simulink model "nms_sim_2D_cost"  (R2024b)
settings: Solver=ode15s  StartTime=0.0  StopTime=t_sim  MaxStep=dt_max  EnableMultiTasking=on
values from neighbouring files (symbols this model uses):
  a_BFSH = param_ctrl(35)*1    [setCtrlPar_optim_CPGreflex2001_2D.m]
  a_GAS = param_ctrl(37)*1    [setCtrlPar_optim_CPGreflex2001_2D.m]
  a_GLU = param_ctrl(31)*1    [setCtrlPar_optim_CPGreflex2001_2D.m]
  a_HAM = param_ctrl(33)*1    [setCtrlPar_optim_CPGreflex2001_2D.m]
  a_HFL = param_ctrl(32)*1    [setCtrlPar_optim_CPGreflex2001_2D.m]
  a_RF = param_ctrl(34)*1    [setCtrlPar_optim_CPGreflex2001_2D.m]
  a_SOL = param_ctrl(38)*1    [setCtrlPar_optim_CPGreflex2001_2D.m]
  a_TA = param_ctrl(39)*1    [setCtrlPar_optim_CPGreflex2001_2D.m]
  a_VAS = param_ctrl(36)*1    [setCtrlPar_optim_CPGreflex2001_2D.m]
  ai = param_ctrl(96)*2.0    [setCtrlPar_optim_CPGreflex2001_2D.m]
  b_BFSH = param_ctrl(52)*.51    [setCtrlPar_optim_CPGreflex2001_2D.m]
  b_BFSHGAS = param_ctrl(55)*.51    [setCtrlPar_optim_CPGreflex2001_2D.m]
  b_BFSHHAM = param_ctrl(54)*.51    [setCtrlPar_optim_CPGreflex2001_2D.m]
  b_BFSHVAS = param_ctrl(53)*.51    [setCtrlPar_optim_CPGreflex2001_2D.m]
  b_GAS = param_ctrl(59)*.51    [setCtrlPar_optim_CPGreflex2001_2D.m]
  b_GASBFSH = param_ctrl(60)*.51    [setCtrlPar_optim_CPGreflex2001_2D.m]
  b_GASSOL = param_ctrl(61)*.51    [setCtrlPar_optim_CPGreflex2001_2D.m]
  b_GLU = param_ctrl(40)*.51    [setCtrlPar_optim_CPGreflex2001_2D.m]
  b_GLUHAM = param_ctrl(42)*.51    [setCtrlPar_optim_CPGreflex2001_2D.m]
  b_GLUHFL = param_ctrl(41)*.51    [setCtrlPar_optim_CPGreflex2001_2D.m]
  b_HAM = param_ctrl(46)*.51    [setCtrlPar_optim_CPGreflex2001_2D.m]
  b_HAMBFSH = param_ctrl(48)*.51    [setCtrlPar_optim_CPGreflex2001_2D.m]
  b_HAMGLU = param_ctrl(47)*.51    [setCtrlPar_optim_CPGreflex2001_2D.m]
  b_HFL = param_ctrl(43)*.51    [setCtrlPar_optim_CPGreflex2001_2D.m]
  b_HFLGLU = param_ctrl(44)*.51    [setCtrlPar_optim_CPGreflex2001_2D.m]
  b_HFLRF = param_ctrl(45)*.51    [setCtrlPar_optim_CPGreflex2001_2D.m]
  b_RF = param_ctrl(49)*.51    [setCtrlPar_optim_CPGreflex2001_2D.m]
  b_RFHFL = param_ctrl(50)*.51    [setCtrlPar_optim_CPGreflex2001_2D.m]
  b_RFVAS = param_ctrl(51)*.51    [setCtrlPar_optim_CPGreflex2001_2D.m]
  b_SOL = param_ctrl(62)*.51    [setCtrlPar_optim_CPGreflex2001_2D.m]
  b_SOLGAS = param_ctrl(64)*.51    [setCtrlPar_optim_CPGreflex2001_2D.m]
  b_SOLTA = param_ctrl(63)*.51    [setCtrlPar_optim_CPGreflex2001_2D.m]
  b_TA = param_ctrl(65)*.51    [setCtrlPar_optim_CPGreflex2001_2D.m]
  b_TASOL = param_ctrl(66)*.51    [setCtrlPar_optim_CPGreflex2001_2D.m]
  b_VAS = param_ctrl(56)*.51    [setCtrlPar_optim_CPGreflex2001_2D.m]
  b_VASBFSH = param_ctrl(57)*.51    [setCtrlPar_optim_CPGreflex2001_2D.m]
  b_VASRF = param_ctrl(58)*.51    [setCtrlPar_optim_CPGreflex2001_2D.m]
  bias = param_ctrl(97)*2.5    [setCtrlPar_optim_CPGreflex2001_2D.m]
  c = 0.05    [nms_MS_2D_scaled.m]
  c_jointstop = 0.3 / (pi/180)    (= 17.1887338539)    [nms_MS_2D_scaled.m]
  D12_F = 0.16    *scaleL_JPhys    [nms_MechInit_2D_scaleSkel.m]
  D12_S = 0.2460	*sub_height    [nms_MechInit_2D_scaleSkel.m]
  D12_T = 0.2450  *sub_height    [nms_MechInit_2D_scaleSkel.m]
  D12y_F = 0.039  *sub_height    [nms_MechInit_2D_scaleSkel.m]
  D12z_HAT = 0.1    [nms_MS_2D_scaled.m]
  D13_F = 0.20    *scaleL_JPhys    [nms_MechInit_2D_scaleSkel.m]
  D1G_F = 0.14    *scaleL_JPhys    [nms_MechInit_2D_scaleSkel.m]
  D1G_HAT = 0.35  *scaleL_JPhys    [nms_MechInit_2D_scaleSkel.m]
  D1G_S = (0.3 - D12y_F/4)	*scaleL_JPhys    [nms_MechInit_2D_scaleSkel.m]
  D1G_T = (0.3 - D12y_F/4)	*scaleL_JPhys    [nms_MechInit_2D_scaleSkel.m]
  D1Gy_F = D12y_F*D1G_F/D12_F    (= 0.07)    [nms_MechInit_2D_scaleSkel.m]
  d_BFSH = param_ctrl(26)*1    [setCtrlPar_optim_CPGreflex2001_2D.m]
  d_GAS = param_ctrl(28)*1    [setCtrlPar_optim_CPGreflex2001_2D.m]
  d_GLU = param_ctrl(22)*1    [setCtrlPar_optim_CPGreflex2001_2D.m]
  d_HAM = param_ctrl(24)*1    [setCtrlPar_optim_CPGreflex2001_2D.m]
  d_HFL = param_ctrl(23)*1    [setCtrlPar_optim_CPGreflex2001_2D.m]
  d_RF = param_ctrl(25)*1    [setCtrlPar_optim_CPGreflex2001_2D.m]
  d_SOL = param_ctrl(29)*1    [setCtrlPar_optim_CPGreflex2001_2D.m]
  d_TA = param_ctrl(30)*1    [setCtrlPar_optim_CPGreflex2001_2D.m]
  d_VAS = param_ctrl(27)*1    [setCtrlPar_optim_CPGreflex2001_2D.m]
  DeltaThRef = 5e-3    (= 0.005)    [nms_MS_2D_scaled.m]
  dloptBFSH = 3.0    (= 3)    [setCtrlPar_optim_CPGreflex2001_2D.m]
  dloptGAS = 3.0    (= 3)    [setCtrlPar_optim_CPGreflex2001_2D.m]
  dloptGLU = 3.0    (= 3)    [setCtrlPar_optim_CPGreflex2001_2D.m]
  dloptHAM = 3.0    (= 3)    [setCtrlPar_optim_CPGreflex2001_2D.m]
  dloptHFL = 3.0    (= 3)    [setCtrlPar_optim_CPGreflex2001_2D.m]
  dloptRF = 3.0    (= 3)    [setCtrlPar_optim_CPGreflex2001_2D.m]
  dloptSOL = 3.0    (= 3)    [setCtrlPar_optim_CPGreflex2001_2D.m]
  dloptTA = 3.0    (= 3)    [setCtrlPar_optim_CPGreflex2001_2D.m]
  dloptVAS = 3.0    (= 3)    [setCtrlPar_optim_CPGreflex2001_2D.m]
  ec_BFSH = param_ctrl(80)*0.15    [setCtrlPar_optim_CPGreflex2001_2D.m]
  ec_GAS = param_ctrl(82)*0.15    [setCtrlPar_optim_CPGreflex2001_2D.m]
  ec_GLU = param_ctrl(76)*0.15    [setCtrlPar_optim_CPGreflex2001_2D.m]
  ec_HAM = param_ctrl(78)*0.15    [setCtrlPar_optim_CPGreflex2001_2D.m]
  ec_HFL = param_ctrl(77)*0.15    [setCtrlPar_optim_CPGreflex2001_2D.m]
  ec_RF = param_ctrl(79)*0.15    [setCtrlPar_optim_CPGreflex2001_2D.m]
  ec_TA = param_ctrl(84)*0.15    [setCtrlPar_optim_CPGreflex2001_2D.m]
  ec_VAS = param_ctrl(81)*0.15    [setCtrlPar_optim_CPGreflex2001_2D.m]
  eref = 0.04    [nms_MS_2D_scaled.m]
  eref_GAS = 0.1    [nms_MS_2D_scaled.m]
  eref_SOL = 0.1    [nms_MS_2D_scaled.m]
  es_BFSH = param_ctrl(89)*0.15    [setCtrlPar_optim_CPGreflex2001_2D.m]
  es_GAS = param_ctrl(91)*0.15    [setCtrlPar_optim_CPGreflex2001_2D.m]
  es_GLU = param_ctrl(85)*0.15    [setCtrlPar_optim_CPGreflex2001_2D.m]
  es_HAM = param_ctrl(87)*0.15    [setCtrlPar_optim_CPGreflex2001_2D.m]
  es_HFL = param_ctrl(86)*0.15    [setCtrlPar_optim_CPGreflex2001_2D.m]
  es_RF = param_ctrl(88)*0.15    [setCtrlPar_optim_CPGreflex2001_2D.m]
  es_TA = param_ctrl(93)*0.15    [setCtrlPar_optim_CPGreflex2001_2D.m]
  es_VAS = param_ctrl(90)*0.15    [setCtrlPar_optim_CPGreflex2001_2D.m]
  FmaxBFSH = 350    [nms_MS_2D_scaled.m]
  FmaxGAS = 2000    [nms_MS_2D_scaled.m]
  FmaxGLU = 4000    [nms_MS_2D_scaled.m]
  FmaxHAM = 2000    [nms_MS_2D_scaled.m]
  FmaxHFL = 2000    [nms_MS_2D_scaled.m]
  FmaxRF = 850    [nms_MS_2D_scaled.m]
  FmaxSOL = 4000    [nms_MS_2D_scaled.m]
  FmaxTA = 800    [nms_MS_2D_scaled.m]
  FmaxVAS = 5000    [nms_MS_2D_scaled.m]
  g = 9.81    [nms_MS_2D_scaled.m]
  gamma_4 = param_ctrl(11) * 1.7    [setCtrlPar_optim_CPGreflexsynergy2023_2D.m]
  h_BFSH = param_ctrl(71)*.1    [setCtrlPar_optim_CPGreflex2001_2D.m]
  h_GAS = param_ctrl(73)*.1    [setCtrlPar_optim_CPGreflex2001_2D.m]
  h_GLU = param_ctrl(67)*.1    [setCtrlPar_optim_CPGreflex2001_2D.m]
  h_HAM = param_ctrl(69)*.1    [setCtrlPar_optim_CPGreflex2001_2D.m]
  h_HFL = param_ctrl(68)*.1    [setCtrlPar_optim_CPGreflex2001_2D.m]
  h_RF = param_ctrl(70)*.1    [setCtrlPar_optim_CPGreflex2001_2D.m]
  h_SOL = param_ctrl(74)*.1    [setCtrlPar_optim_CPGreflex2001_2D.m]
  h_TA = param_ctrl(75)*.1    [setCtrlPar_optim_CPGreflex2001_2D.m]
  h_VAS = param_ctrl(72)*.1    [setCtrlPar_optim_CPGreflex2001_2D.m]
  HLCtrlPar = [theta_tgt l_clr alpha_tgt alpha_cd alpha_cv]    [setCtrlPar_optim_reflex2015_2D.m]
  In_F = 0.005    *scaleM*scaleL_JPhys^2    [nms_MechInit_2D_scaleSkel.m]
  In_HAT = 2.5    *scaleM*scaleL_JPhys^2    [nms_MechInit_2D_scaleSkel.m]
  In_S = 0.05     *scaleM*scaleL_JPhys^2    [nms_MechInit_2D_scaleSkel.m]
  In_T = 0.15     *scaleM*scaleL_JPhys^2    [nms_MechInit_2D_scaleSkel.m]
  init_exc = 0.01    [setInitPar_optim_2D.m]
  init_fm = 0.01    [setInitPar_optim_2D.m]
  init_lce = 1    [setInitPar_optim_2D.m]
  init_LCPG = param_ctrl(12) * 0.01    [setCtrlPar_optim_CPGreflexsynergy2023_2D.m]
  init_LStance = 1    [setInitPar_optim_2D.m]
  init_N1 = osc_signal1(phi_off_osc_ind)    [setCtrlPar_optim_CPGreflex2001_2D.m]
  ... (+441 more)
undefined symbols (not defined in the file or in its folder): cost_act_exponent, cost_v_tgt, flag_controller, Newton, nStep_obj, nStep_startKin, Raphson, sgn, SSW_kin, terrain_slope_angle, v_plateS1, X, Y, Z
libraries: nesl_utility x94, sm_lib x90, simulink x28, simulink_extras x12
(part 7 of 20)

== system nms_sim_2D_cost/CPG-reflex Controller/Muscle Spindle GLU ==
  note: Lm
  Lce : Inport
  Vce : Inport  Port=2
  Constant2 : Constant
  Constant3 : Constant  Value=0
  Constant4 : Constant
  Gain2 : Gain  Gain=1/tao_spindle
  Gain3 : Gain  Gain=p_GLU
  Gain4 : Gain  Gain=q_GLU
  GreaterThan : RelationalOperator  OutDataTypeStr=boolean  RndMeth=Simplest  InputSameDT=off
  Integrator : Integrator  InitialCondition=init_lce
  Saturation : Saturate  UpperLimit=inf  LowerLimit=0
  Saturation1 : Saturate  UpperLimit=inf  LowerLimit=0
  Saturation2 : Saturate  UpperLimit=inf  LowerLimit=0
  Sum4 : Sum  Inputs=|+-
  Sum5 : Sum  Inputs=-++
  Switch : Switch  Criteria=u2 > Threshold  SaturateOnIntegerOverflow=off  InputSameDT=off
  Sm : Outport
  wires:
  Constant2/1 -> Sum4/2
  Saturation/1 -> Gain4/1
  Constant3/1 -> Switch/3
  Constant4/1 -> GreaterThan/2
  GreaterThan/1 -> Switch/2
  Switch/1 -> Sm/1  "Sm"
  Saturation2/1 -> Switch/1
  Gain2/1 -> Integrator/1
  Lce/1 -> Sum4/1, GreaterThan/1  "Lm"
  Saturation1/1 -> Gain3/1
  Gain4/1 -> Sum5/2
  Sum5/1 -> Saturation2/1, Gain2/1
  Integrator/1 -> Sum5/1
  Gain3/1 -> Sum5/3
  Sum4/1 -> Saturation/1
  Vce/1 -> Saturation1/1  "vm"

== system nms_sim_2D_cost/CPG-reflex Controller/Muscle Spindle GLU2 ==
  note: Lm
  Lce : Inport
  Vce : Inport  Port=2
  Constant2 : Constant
  Constant3 : Constant  Value=0
  Constant4 : Constant
  Gain2 : Gain  Gain=1/tao_spindle
  Gain3 : Gain  Gain=p_GLU
  Gain4 : Gain  Gain=q_GLU
  GreaterThan : RelationalOperator  OutDataTypeStr=boolean  RndMeth=Simplest  InputSameDT=off
  Integrator : Integrator  InitialCondition=init_lce
  Saturation : Saturate  UpperLimit=inf  LowerLimit=0
  Saturation1 : Saturate  UpperLimit=inf  LowerLimit=0
  Saturation2 : Saturate  UpperLimit=inf  LowerLimit=0
  Sum4 : Sum  Inputs=|+-
  Sum5 : Sum  Inputs=-++
  Switch : Switch  Criteria=u2 > Threshold  SaturateOnIntegerOverflow=off  InputSameDT=off
  Sm : Outport
  wires:
  Constant2/1 -> Sum4/2
  Saturation/1 -> Gain4/1
  Constant3/1 -> Switch/3
  Constant4/1 -> GreaterThan/2
  GreaterThan/1 -> Switch/2
  Switch/1 -> Sm/1  "Sm"
  Saturation2/1 -> Switch/1
  Gain2/1 -> Integrator/1
  Lce/1 -> Sum4/1, GreaterThan/1  "Lm"
  Saturation1/1 -> Gain3/1
  Gain4/1 -> Sum5/2
  Sum5/1 -> Saturation2/1, Gain2/1
  Integrator/1 -> Sum5/1
  Gain3/1 -> Sum5/3
  Sum4/1 -> Saturation/1
  Vce/1 -> Saturation1/1  "vm"

== system nms_sim_2D_cost/CPG-reflex Controller/Muscle Spindle HAM ==
  note: Lm
  Lce : Inport
  Vce : Inport  Port=2
  Constant2 : Constant
  Constant3 : Constant  Value=0
  Constant4 : Constant
  Gain2 : Gain  Gain=1/tao_spindle
  Gain3 : Gain  Gain=p_HAM
  Gain4 : Gain  Gain=q_HAM
  GreaterThan : RelationalOperator  OutDataTypeStr=boolean  RndMeth=Simplest  InputSameDT=off
  Integrator : Integrator  InitialCondition=init_lce
  Saturation : Saturate  UpperLimit=inf  LowerLimit=0
  Saturation1 : Saturate  UpperLimit=inf  LowerLimit=0
  Saturation2 : Saturate  UpperLimit=inf  LowerLimit=0
  Sum4 : Sum  Inputs=|+-
  Sum5 : Sum  Inputs=-++
  Switch : Switch  Criteria=u2 > Threshold  SaturateOnIntegerOverflow=off  InputSameDT=off
  Sm : Outport
  wires:
  Constant2/1 -> Sum4/2
  Saturation/1 -> Gain4/1
  Constant3/1 -> Switch/3
  Constant4/1 -> GreaterThan/2
  GreaterThan/1 -> Switch/2
  Switch/1 -> Sm/1  "Sm"
  Saturation2/1 -> Switch/1
  Gain2/1 -> Integrator/1
  Lce/1 -> Sum4/1, GreaterThan/1  "Lm"
  Saturation1/1 -> Gain3/1
  Gain4/1 -> Sum5/2
  Sum5/1 -> Saturation2/1, Gain2/1
  Integrator/1 -> Sum5/1
  Gain3/1 -> Sum5/3
  Sum4/1 -> Saturation/1
  Vce/1 -> Saturation1/1  "vm"

== system nms_sim_2D_cost/CPG-reflex Controller/Muscle Spindle HAM2 ==
  note: Lm
  Lce : Inport
  Vce : Inport  Port=2
  Constant2 : Constant
  Constant3 : Constant  Value=0
  Constant4 : Constant
  Gain2 : Gain  Gain=1/tao_spindle
  Gain3 : Gain  Gain=p_HAM
  Gain4 : Gain  Gain=q_HAM
  GreaterThan : RelationalOperator  OutDataTypeStr=boolean  RndMeth=Simplest  InputSameDT=off
  Integrator : Integrator  InitialCondition=init_lce
  Saturation : Saturate  UpperLimit=inf  LowerLimit=0
  Saturation1 : Saturate  UpperLimit=inf  LowerLimit=0
  Saturation2 : Saturate  UpperLimit=inf  LowerLimit=0
  Sum4 : Sum  Inputs=|+-
  Sum5 : Sum  Inputs=-++
  Switch : Switch  Criteria=u2 > Threshold  SaturateOnIntegerOverflow=off  InputSameDT=off
  Sm : Outport
  wires:
  Constant2/1 -> Sum4/2
  Saturation/1 -> Gain4/1
  Constant3/1 -> Switch/3
  Constant4/1 -> GreaterThan/2
  GreaterThan/1 -> Switch/2
  Switch/1 -> Sm/1  "Sm"
  Saturation2/1 -> Switch/1
  Gain2/1 -> Integrator/1
  Lce/1 -> Sum4/1, GreaterThan/1  "Lm"
  Saturation1/1 -> Gain3/1
  Gain4/1 -> Sum5/2
  Sum5/1 -> Saturation2/1, Gain2/1
  Integrator/1 -> Sum5/1
  Gain3/1 -> Sum5/3
  Sum4/1 -> Saturation/1
  Vce/1 -> Saturation1/1  "vm"

== system nms_sim_2D_cost/CPG-reflex Controller/Muscle Spindle HFL ==
  note: Lm
  Lce : Inport
  Vce : Inport  Port=2
  Constant2 : Constant
  Constant3 : Constant  Value=0
  Constant4 : Constant
  Gain2 : Gain  Gain=1/tao_spindle
  Gain3 : Gain  Gain=p_HFL
  Gain4 : Gain  Gain=q_HFL
  GreaterThan : RelationalOperator  OutDataTypeStr=boolean  RndMeth=Simplest  InputSameDT=off
  Integrator : Integrator  InitialCondition=init_lce
  Saturation : Saturate  UpperLimit=inf  LowerLimit=0
  Saturation1 : Saturate  UpperLimit=inf  LowerLimit=0
  Saturation2 : Saturate  UpperLimit=inf  LowerLimit=0
  Sum4 : Sum  Inputs=|+-
  Sum5 : Sum  Inputs=-++
  Switch : Switch  Criteria=u2 > Threshold  SaturateOnIntegerOverflow=off  InputSameDT=off
  Sm : Outport
  wires:
  Constant2/1 -> Sum4/2
  Saturation/1 -> Gain4/1
  Constant3/1 -> Switch/3
  Constant4/1 -> GreaterThan/2
  GreaterThan/1 -> Switch/2
  Switch/1 -> Sm/1  "Sm"
  Saturation2/1 -> Switch/1
  Gain2/1 -> Integrator/1
  Lce/1 -> Sum4/1, GreaterThan/1  "Lm"
  Saturation1/1 -> Gain3/1
  Gain4/1 -> Sum5/2
  Sum5/1 -> Saturation2/1, Gain2/1
  Integrator/1 -> Sum5/1
  Gain3/1 -> Sum5/3
  Sum4/1 -> Saturation/1
  Vce/1 -> Saturation1/1  "vm"

== system nms_sim_2D_cost/CPG-reflex Controller/Muscle Spindle HFL2 ==
  note: Lm
  Lce : Inport
  Vce : Inport  Port=2
  Constant2 : Constant
  Constant3 : Constant  Value=0
  Constant4 : Constant
  Gain2 : Gain  Gain=1/tao_spindle
  Gain3 : Gain  Gain=p_HFL
  Gain4 : Gain  Gain=q_HFL
  GreaterThan : RelationalOperator  OutDataTypeStr=boolean  RndMeth=Simplest  InputSameDT=off
  Integrator : Integrator  InitialCondition=init_lce
  Saturation : Saturate  UpperLimit=inf  LowerLimit=0
  Saturation1 : Saturate  UpperLimit=inf  LowerLimit=0
  Saturation2 : Saturate  UpperLimit=inf  LowerLimit=0
  Sum4 : Sum  Inputs=|+-
  Sum5 : Sum  Inputs=-++
  Switch : Switch  Criteria=u2 > Threshold  SaturateOnIntegerOverflow=off  InputSameDT=off
  Sm : Outport
  wires:
  Constant2/1 -> Sum4/2
  Saturation/1 -> Gain4/1
  Constant3/1 -> Switch/3
  Constant4/1 -> GreaterThan/2
  GreaterThan/1 -> Switch/2
  Switch/1 -> Sm/1  "Sm"
  Saturation2/1 -> Switch/1
  Gain2/1 -> Integrator/1
  Lce/1 -> Sum4/1, GreaterThan/1  "Lm"
  Saturation1/1 -> Gain3/1
  Gain4/1 -> Sum5/2
  Sum5/1 -> Saturation2/1, Gain2/1
  Integrator/1 -> Sum5/1
  Gain3/1 -> Sum5/3
  Sum4/1 -> Saturation/1
  Vce/1 -> Saturation1/1  "vm"

== system nms_sim_2D_cost/CPG-reflex Controller/Muscle Spindle RF ==
  note: Lm
  Lce : Inport
  Vce : Inport  Port=2
  Constant2 : Constant
  Constant3 : Constant  Value=0
  Constant4 : Constant
  Gain2 : Gain  Gain=1/tao_spindle
  Gain3 : Gain  Gain=p_RF
  Gain4 : Gain  Gain=q_RF
  GreaterThan : RelationalOperator  OutDataTypeStr=boolean  RndMeth=Simplest  InputSameDT=off
  Integrator : Integrator  InitialCondition=init_lce
  Saturation : Saturate  UpperLimit=inf  LowerLimit=0
  Saturation1 : Saturate  UpperLimit=inf  LowerLimit=0
  Saturation2 : Saturate  UpperLimit=inf  LowerLimit=0
  Sum4 : Sum  Inputs=|+-
  Sum5 : Sum  Inputs=-++
  Switch : Switch  Criteria=u2 > Threshold  SaturateOnIntegerOverflow=off  InputSameDT=off
  Sm : Outport
  wires:
  Constant2/1 -> Sum4/2
  Saturation/1 -> Gain4/1
  Constant3/1 -> Switch/3
  Constant4/1 -> GreaterThan/2
  GreaterThan/1 -> Switch/2
  Switch/1 -> Sm/1  "Sm"
  Saturation2/1 -> Switch/1
  Gain2/1 -> Integrator/1
  Lce/1 -> Sum4/1, GreaterThan/1  "Lm"
  Saturation1/1 -> Gain3/1
  Gain4/1 -> Sum5/2
  Sum5/1 -> Saturation2/1, Gain2/1
  Integrator/1 -> Sum5/1
  Gain3/1 -> Sum5/3
  Sum4/1 -> Saturation/1
  Vce/1 -> Saturation1/1  "vm"

== system nms_sim_2D_cost/CPG-reflex Controller/Muscle Spindle RF2 ==
  note: Lm
  Lce : Inport
  Vce : Inport  Port=2
  Constant2 : Constant
  Constant3 : Constant  Value=0
  Constant4 : Constant
  Gain2 : Gain  Gain=1/tao_spindle
  Gain3 : Gain  Gain=p_RF
  Gain4 : Gain  Gain=q_RF
  GreaterThan : RelationalOperator  OutDataTypeStr=boolean  RndMeth=Simplest  InputSameDT=off
  Integrator : Integrator  InitialCondition=init_lce
  Saturation : Saturate  UpperLimit=inf  LowerLimit=0
  Saturation1 : Saturate  UpperLimit=inf  LowerLimit=0
  Saturation2 : Saturate  UpperLimit=inf  LowerLimit=0
  Sum4 : Sum  Inputs=|+-
  Sum5 : Sum  Inputs=-++
  Switch : Switch  Criteria=u2 > Threshold  SaturateOnIntegerOverflow=off  InputSameDT=off
  Sm : Outport
  wires:
  Constant2/1 -> Sum4/2
  Saturation/1 -> Gain4/1
  Constant3/1 -> Switch/3
  Constant4/1 -> GreaterThan/2
  GreaterThan/1 -> Switch/2
  Switch/1 -> Sm/1  "Sm"
  Saturation2/1 -> Switch/1
  Gain2/1 -> Integrator/1
  Lce/1 -> Sum4/1, GreaterThan/1  "Lm"
  Saturation1/1 -> Gain3/1
  Gain4/1 -> Sum5/2
  Sum5/1 -> Saturation2/1, Gain2/1
  Integrator/1 -> Sum5/1
  Gain3/1 -> Sum5/3
  Sum4/1 -> Saturation/1
  Vce/1 -> Saturation1/1  "vm"

== system nms_sim_2D_cost/CPG-reflex Controller/Muscle Spindle SOL ==
  note: Lm
  Lce : Inport
  Vce : Inport  Port=2
  Constant2 : Constant
  Constant3 : Constant  Value=0
  Constant4 : Constant
  Gain2 : Gain  Gain=1/tao_spindle
  Gain3 : Gain  Gain=p_SOL
  Gain4 : Gain  Gain=q_SOL
  GreaterThan : RelationalOperator  OutDataTypeStr=boolean  RndMeth=Simplest  InputSameDT=off
  Integrator : Integrator  InitialCondition=init_lce
  Saturation : Saturate  UpperLimit=inf  LowerLimit=0
  Saturation1 : Saturate  UpperLimit=inf  LowerLimit=0
  Saturation2 : Saturate  UpperLimit=inf  LowerLimit=0
  Sum4 : Sum  Inputs=|+-
  Sum5 : Sum  Inputs=-++
  Switch : Switch  Criteria=u2 > Threshold  SaturateOnIntegerOverflow=off  InputSameDT=off
  Sm : Outport
  wires:
  Constant2/1 -> Sum4/2
  Saturation/1 -> Gain4/1
  Constant3/1 -> Switch/3
  Constant4/1 -> GreaterThan/2
  GreaterThan/1 -> Switch/2
  Switch/1 -> Sm/1  "Sm"
  Saturation2/1 -> Switch/1
  Gain2/1 -> Integrator/1
  Lce/1 -> Sum4/1, GreaterThan/1  "Lm"
  Saturation1/1 -> Gain3/1
  Gain4/1 -> Sum5/2
  Sum5/1 -> Saturation2/1, Gain2/1
  Integrator/1 -> Sum5/1
  Gain3/1 -> Sum5/3
  Sum4/1 -> Saturation/1
  Vce/1 -> Saturation1/1  "vm"

== system nms_sim_2D_cost/CPG-reflex Controller/Muscle Spindle SOL2 ==
  note: Lm
  Lce : Inport
  Vce : Inport  Port=2
  Constant2 : Constant
  Constant3 : Constant  Value=0
  Constant4 : Constant
  Gain2 : Gain  Gain=1/tao_spindle
  Gain3 : Gain  Gain=p_SOL
  Gain4 : Gain  Gain=q_SOL
  GreaterThan : RelationalOperator  OutDataTypeStr=boolean  RndMeth=Simplest  InputSameDT=off
  Integrator : Integrator  InitialCondition=init_lce
  Saturation : Saturate  UpperLimit=inf  LowerLimit=0
  Saturation1 : Saturate  UpperLimit=inf  LowerLimit=0
  Saturation2 : Saturate  UpperLimit=inf  LowerLimit=0
  Sum4 : Sum  Inputs=|+-
  Sum5 : Sum  Inputs=-++
  Switch : Switch  Criteria=u2 > Threshold  SaturateOnIntegerOverflow=off  InputSameDT=off
  Sm : Outport
  wires:
  Constant2/1 -> Sum4/2
  Saturation/1 -> Gain4/1
  Constant3/1 -> Switch/3
  Constant4/1 -> GreaterThan/2
  GreaterThan/1 -> Switch/2
  Switch/1 -> Sm/1  "Sm"
  Saturation2/1 -> Switch/1
  Gain2/1 -> Integrator/1
  Lce/1 -> Sum4/1, GreaterThan/1  "Lm"
  Saturation1/1 -> Gain3/1
  Gain4/1 -> Sum5/2
  Sum5/1 -> Saturation2/1, Gain2/1
  Integrator/1 -> Sum5/1
  Gain3/1 -> Sum5/3
  Sum4/1 -> Saturation/1
  Vce/1 -> Saturation1/1  "vm"

== system nms_sim_2D_cost/CPG-reflex Controller/Muscle Spindle TA ==
  note: Lm
  Lce : Inport
  Vce : Inport  Port=2
  Constant2 : Constant
  Constant3 : Constant  Value=0
  Constant4 : Constant
  Gain2 : Gain  Gain=1/tao_spindle
  Gain3 : Gain  Gain=p_TA
  Gain4 : Gain  Gain=q_TA
  GreaterThan : RelationalOperator  OutDataTypeStr=boolean  RndMeth=Simplest  InputSameDT=off
  Integrator : Integrator  InitialCondition=init_lce
  Saturation : Saturate  UpperLimit=inf  LowerLimit=0
  Saturation1 : Saturate  UpperLimit=inf  LowerLimit=0
  Saturation2 : Saturate  UpperLimit=inf  LowerLimit=0
  Sum4 : Sum  Inputs=|+-
  Sum5 : Sum  Inputs=-++
  Switch : Switch  Criteria=u2 > Threshold  SaturateOnIntegerOverflow=off  InputSameDT=off
  Sm : Outport
  wires:
  Constant2/1 -> Sum4/2
  Saturation/1 -> Gain4/1
  Constant3/1 -> Switch/3
  Constant4/1 -> GreaterThan/2
  GreaterThan/1 -> Switch/2
  Switch/1 -> Sm/1  "Sm"
  Saturation2/1 -> Switch/1
  Gain2/1 -> Integrator/1
  Lce/1 -> Sum4/1, GreaterThan/1  "Lm"
  Saturation1/1 -> Gain3/1
  Gain4/1 -> Sum5/2
  Sum5/1 -> Saturation2/1, Gain2/1
  Integrator/1 -> Sum5/1
  Gain3/1 -> Sum5/3
  Sum4/1 -> Saturation/1
  Vce/1 -> Saturation1/1  "vm"

== system nms_sim_2D_cost/CPG-reflex Controller/Muscle Spindle TA2 ==
  note: Lm
  Lce : Inport
  Vce : Inport  Port=2
  Constant2 : Constant
  Constant3 : Constant  Value=0
  Constant4 : Constant
  Gain2 : Gain  Gain=1/tao_spindle
  Gain3 : Gain  Gain=p_TA
  Gain4 : Gain  Gain=q_TA
  GreaterThan : RelationalOperator  OutDataTypeStr=boolean  RndMeth=Simplest  InputSameDT=off
  Integrator : Integrator  InitialCondition=init_lce
  Saturation : Saturate  UpperLimit=inf  LowerLimit=0
  Saturation1 : Saturate  UpperLimit=inf  LowerLimit=0
  Saturation2 : Saturate  UpperLimit=inf  LowerLimit=0
  Sum4 : Sum  Inputs=|+-
  Sum5 : Sum  Inputs=-++
  Switch : Switch  Criteria=u2 > Threshold  SaturateOnIntegerOverflow=off  InputSameDT=off
  Sm : Outport
  wires:
  Constant2/1 -> Sum4/2
  Saturation/1 -> Gain4/1
  Constant3/1 -> Switch/3
  Constant4/1 -> GreaterThan/2
  GreaterThan/1 -> Switch/2
  Switch/1 -> Sm/1  "Sm"
  Saturation2/1 -> Switch/1
  Gain2/1 -> Integrator/1
  Lce/1 -> Sum4/1, GreaterThan/1  "Lm"
  Saturation1/1 -> Gain3/1
  Gain4/1 -> Sum5/2
  Sum5/1 -> Saturation2/1, Gain2/1
  Integrator/1 -> Sum5/1
  Gain3/1 -> Sum5/3
  Sum4/1 -> Saturation/1
  Vce/1 -> Saturation1/1  "vm"

== system nms_sim_2D_cost/CPG-reflex Controller/Muscle Spindle VAS ==
  note: Lm
  Lce : Inport
  Vce : Inport  Port=2
  Constant2 : Constant
  Constant3 : Constant  Value=0
  Constant4 : Constant
  Gain2 : Gain  Gain=1/tao_spindle
  Gain3 : Gain  Gain=p_VAS
  Gain4 : Gain  Gain=q_VAS
  GreaterThan : RelationalOperator  OutDataTypeStr=boolean  RndMeth=Simplest  InputSameDT=off
  Integrator : Integrator  InitialCondition=init_lce
  Saturation : Saturate  UpperLimit=inf  LowerLimit=0
  Saturation1 : Saturate  UpperLimit=inf  LowerLimit=0
  Saturation2 : Saturate  UpperLimit=inf  LowerLimit=0
  Sum4 : Sum  Inputs=|+-
  Sum5 : Sum  Inputs=-++
  Switch : Switch  Criteria=u2 > Threshold  SaturateOnIntegerOverflow=off  InputSameDT=off
  Sm : Outport
  wires:
  Constant2/1 -> Sum4/2
  Saturation/1 -> Gain4/1
  Constant3/1 -> Switch/3
  Constant4/1 -> GreaterThan/2
  GreaterThan/1 -> Switch/2
  Switch/1 -> Sm/1  "Sm"
  Saturation2/1 -> Switch/1
  Gain2/1 -> Integrator/1
  Lce/1 -> Sum4/1, GreaterThan/1  "Lm"
  Saturation1/1 -> Gain3/1
  Gain4/1 -> Sum5/2
  Sum5/1 -> Saturation2/1, Gain2/1
  Integrator/1 -> Sum5/1
  Gain3/1 -> Sum5/3
  Sum4/1 -> Saturation/1
  Vce/1 -> Saturation1/1  "vm"

== system nms_sim_2D_cost/CPG-reflex Controller/Muscle Spindle VAS2 ==
  note: Lm
  Lce : Inport
  Vce : Inport  Port=2
  Constant2 : Constant
  Constant3 : Constant  Value=0
  Constant4 : Constant
  Gain2 : Gain  Gain=1/tao_spindle
  Gain3 : Gain  Gain=p_VAS
  Gain4 : Gain  Gain=q_VAS
  GreaterThan : RelationalOperator  OutDataTypeStr=boolean  RndMeth=Simplest  InputSameDT=off
  Integrator : Integrator  InitialCondition=init_lce
  Saturation : Saturate  UpperLimit=inf  LowerLimit=0
  Saturation1 : Saturate  UpperLimit=inf  LowerLimit=0
  Saturation2 : Saturate  UpperLimit=inf  LowerLimit=0
  Sum4 : Sum  Inputs=|+-
  Sum5 : Sum  Inputs=-++
  Switch : Switch  Criteria=u2 > Threshold  SaturateOnIntegerOverflow=off  InputSameDT=off
  Sm : Outport
  wires:
  Constant2/1 -> Sum4/2
  Saturation/1 -> Gain4/1
  Constant3/1 -> Switch/3
  Constant4/1 -> GreaterThan/2
  GreaterThan/1 -> Switch/2
  Switch/1 -> Sm/1  "Sm"
  Saturation2/1 -> Switch/1
  Gain2/1 -> Integrator/1
  Lce/1 -> Sum4/1, GreaterThan/1  "Lm"
  Saturation1/1 -> Gain3/1
  Gain4/1 -> Sum5/2
  Sum5/1 -> Saturation2/1, Gain2/1
  Integrator/1 -> Sum5/1
  Gain3/1 -> Sum5/3
  Sum4/1 -> Saturation/1
  Vce/1 -> Saturation1/1  "vm"

== system nms_sim_2D_cost/CPG-reflex Controller/feedback ==
  LStance : Inport
  Constant : Constant
  Gain : Gain  Gain=ec_GLU
  Gain1 : Gain  Gain=es_GLU
  Sum : Sum  Inputs=|-+
  Sum1 : Sum  Inputs=|++
  Feedback : Outport
  wires:
  LStance/1 -> Sum/1, Gain/1
  Constant/1 -> Sum/2
  Gain/1 -> Sum1/1
  Sum1/1 -> Feedback/1
  Sum/1 -> Gain1/1
  Gain1/1 -> Sum1/2

== system nms_sim_2D_cost/CPG-reflex Controller/feedback BFSH ==
  LStance : Inport
  Constant : Constant
  Gain : Gain  Gain=ec_BFSH
  Gain1 : Gain  Gain=es_BFSH
  Sum : Sum  Inputs=|-+
  Sum1 : Sum  Inputs=|++
  FBBFSH : Outport
  wires:
  Gain1/1 -> Sum1/2
  Sum/1 -> Gain1/1
  Sum1/1 -> FBBFSH/1
  Gain/1 -> Sum1/1
  Constant/1 -> Sum/2
  LStance/1 -> Gain/1, Sum/1

== system nms_sim_2D_cost/CPG-reflex Controller/feedback BFSH2 ==
  RStance : Inport
  Constant : Constant
  Gain : Gain  Gain=ec_BFSH
  Gain1 : Gain  Gain=es_BFSH
  Sum : Sum  Inputs=|-+
  Sum1 : Sum  Inputs=|++
  FBBFSH : Outport
  wires:
  RStance/1 -> Sum/1, Gain/1
  Constant/1 -> Sum/2
  Gain/1 -> Sum1/1
  Sum1/1 -> FBBFSH/1
  Sum/1 -> Gain1/1
  Gain1/1 -> Sum1/2

== system nms_sim_2D_cost/CPG-reflex Controller/feedback HFL ==
  LStance : Inport
  Constant : Constant
  Gain : Gain  Gain=ec_HFL
  Gain1 : Gain  Gain=es_HFL
  Sum : Sum  Inputs=|-+
  Sum1 : Sum  Inputs=|++
  FBHFL : Outport
  wires:
  Gain1/1 -> Sum1/2
  Sum/1 -> Gain1/1
  Sum1/1 -> FBHFL/1
  Gain/1 -> Sum1/1
  Constant/1 -> Sum/2
  LStance/1 -> Gain/1, Sum/1

== system nms_sim_2D_cost/CPG-reflex Controller/feedback HFL2 ==
  RStance : Inport
  Constant : Constant
  Gain : Gain  Gain=ec_HFL
  Gain1 : Gain  Gain=es_HFL
  Sum : Sum  Inputs=|-+
  Sum1 : Sum  Inputs=|++
  FBHFL : Outport
  wires:
  RStance/1 -> Sum/1, Gain/1
  Constant/1 -> Sum/2
  Gain/1 -> Sum1/1
  Sum1/1 -> FBHFL/1
  Sum/1 -> Gain1/1
  Gain1/1 -> Sum1/2

== system nms_sim_2D_cost/CPG-reflex Controller/feedback RF ==
  LStance : Inport
  Constant : Constant
  Gain : Gain  Gain=ec_RF
  Gain1 : Gain  Gain=es_RF
  Sum : Sum  Inputs=|-+
  Sum1 : Sum  Inputs=|++
  Feedback : Outport
  wires:
  Gain1/1 -> Sum1/2
  Sum/1 -> Gain1/1
  Sum1/1 -> Feedback/1
  Gain/1 -> Sum1/1
  Constant/1 -> Sum/2
  LStance/1 -> Gain/1, Sum/1

== system nms_sim_2D_cost/CPG-reflex Controller/feedback RF2 ==
  RStance : Inport
  Constant : Constant
  Gain : Gain  Gain=ec_RF
  Gain1 : Gain  Gain=es_RF
  Sum : Sum  Inputs=|-+
  Sum1 : Sum  Inputs=|++
  Feedback : Outport
  wires:
  RStance/1 -> Sum/1, Gain/1
  Constant/1 -> Sum/2
  Gain/1 -> Sum1/1
  Sum1/1 -> Feedback/1
  Sum/1 -> Gain1/1
  Gain1/1 -> Sum1/2

== system nms_sim_2D_cost/CPG-reflex Controller/feedback SOL ==
  LStance : Inport
  Constant : Constant
  Gain : Gain  Gain=ec_GLU
  Gain1 : Gain  Gain=es_GLU
  Sum : Sum  Inputs=|-+
  Sum1 : Sum  Inputs=|++
  FB SOL : Outport
  wires:
  LStance/1 -> Sum/1, Gain/1
  Constant/1 -> Sum/2
  Gain/1 -> Sum1/1
  Sum1/1 -> FB SOL/1
  Sum/1 -> Gain1/1
  Gain1/1 -> Sum1/2

== system nms_sim_2D_cost/CPG-reflex Controller/feedback SOL2 ==
  RStance : Inport
  Constant : Constant
  Gain : Gain  Gain=ec_GLU
  Gain1 : Gain  Gain=es_GLU
  Sum : Sum  Inputs=|-+
  Sum1 : Sum  Inputs=|++
  FB SOL : Outport
  wires:
  Gain1/1 -> Sum1/2
  Sum/1 -> Gain1/1
  Sum1/1 -> FB SOL/1
  Gain/1 -> Sum1/1
  Constant/1 -> Sum/2
  RStance/1 -> Gain/1, Sum/1

== system nms_sim_2D_cost/CPG-reflex Controller/feedback TA ==
  LStance : Inport
  Constant : Constant
  Gain : Gain  Gain=ec_TA
  Gain1 : Gain  Gain=es_TA
  Sum : Sum  Inputs=|-+
  Sum1 : Sum  Inputs=|++
  FB TA : Outport
  wires:
  Gain1/1 -> Sum1/2
  Sum/1 -> Gain1/1
  Sum1/1 -> FB TA/1
  Gain/1 -> Sum1/1
  Constant/1 -> Sum/2
  LStance/1 -> Gain/1, Sum/1

== system nms_sim_2D_cost/CPG-reflex Controller/feedback TA2 ==
  RStance : Inport
  Constant : Constant
  Gain : Gain  Gain=ec_TA
  Gain1 : Gain  Gain=es_TA
  Sum : Sum  Inputs=|-+
  Sum1 : Sum  Inputs=|++
  FB TA : Outport
  wires:
  RStance/1 -> Sum/1, Gain/1
  Constant/1 -> Sum/2
  Gain/1 -> Sum1/1
  Sum1/1 -> FB TA/1
  Sum/1 -> Gain1/1
  Gain1/1 -> Sum1/2

== system nms_sim_2D_cost/CPG-reflex Controller/feedback2 ==
  RStance : Inport
  Constant : Constant
  Gain : Gain  Gain=ec_GLU
  Gain1 : Gain  Gain=es_GLU
  Sum : Sum  Inputs=|-+
  Sum1 : Sum  Inputs=|++
  Feedback : Outport
  wires:
  Gain1/1 -> Sum1/2
  Sum/1 -> Gain1/1
  Sum1/1 -> Feedback/1
  Gain/1 -> Sum1/1
  Constant/1 -> Sum/2
  RStance/1 -> Gain/1, Sum/1

== system nms_sim_2D_cost/CPG-reflex Controller/feedbackGAS ==
  LStance : Inport
  Constant : Constant
  Gain : Gain  Gain=ec_GAS
  Gain1 : Gain  Gain=es_GAS
  Sum : Sum  Inputs=|-+
  Sum1 : Sum  Inputs=|++
  FB GAS : Outport
  wires:
  Gain1/1 -> Sum1/2
  Sum/1 -> Gain1/1
  Sum1/1 -> FB GAS/1
  Gain/1 -> Sum1/1
  Constant/1 -> Sum/2
  LStance/1 -> Gain/1, Sum/1

== system nms_sim_2D_cost/CPG-reflex Controller/feedbackGAS2 ==
  RStance : Inport
  Constant : Constant
  Gain : Gain  Gain=ec_GAS
  Gain1 : Gain  Gain=es_GAS
  Sum : Sum  Inputs=|-+
  Sum1 : Sum  Inputs=|++
  FB GAS : Outport
  wires:
  RStance/1 -> Sum/1, Gain/1
  Constant/1 -> Sum/2
  Gain/1 -> Sum1/1
  Sum1/1 -> FB GAS/1
  Sum/1 -> Gain1/1
  Gain1/1 -> Sum1/2

== system nms_sim_2D_cost/CPG-reflex-synergy controller/Balance Control System GLU ==
  d_theta : Inport
  d_dtheta : Inport  Port=2
  Constant : Constant  Value=tgt_theta_4_GLU
  Gain : Gain  Gain=kp_4_GLU
  Gain1 : Gain  Gain=kv_4_GLU
  Sum : Sum  Inputs=|+-
  Sum1 : Sum  Inputs=|++
  ubalance : Outport
  wires:
  d_theta/1 -> Sum/1
  Constant/1 -> Sum/2
  Sum/1 -> Gain/1
  d_dtheta/1 -> Gain1/1
  Sum1/1 -> ubalance/1
  Gain/1 -> Sum1/1
  Gain1/1 -> Sum1/2

== system nms_sim_2D_cost/CPG-reflex-synergy controller/Balance Control System HAM ==
  d_theta : Inport
  d_dtheta : Inport  Port=2
  Constant : Constant  Value=tgt_theta_4_HAM
  Gain : Gain  Gain=kp_4_HAM
  Gain1 : Gain  Gain=kv_4_HAM
  Sum : Sum  Inputs=|+-
  Sum1 : Sum  Inputs=|++
  ubalance : Outport
  wires:
  Gain1/1 -> Sum1/2
  Gain/1 -> Sum1/1
  Sum1/1 -> ubalance/1
  d_dtheta/1 -> Gain1/1
  Sum/1 -> Gain/1
  Constant/1 -> Sum/2
  d_theta/1 -> Sum/1

== system nms_sim_2D_cost/CPG-reflex-synergy controller/Balance Control System HFL ==
  d_theta : Inport
  d_dtheta : Inport  Port=2
  Constant : Constant  Value=tgt_theta_4_HFL
  Gain : Gain  Gain=kp_4_HFL
  Gain1 : Gain  Gain=kv_4_HFL
  Sum : Sum  Inputs=|+-
  Sum1 : Sum  Inputs=|++
  ubalance : Outport
  wires:
  d_theta/1 -> Sum/1
  Constant/1 -> Sum/2
  Sum/1 -> Gain/1
  d_dtheta/1 -> Gain1/1
  Sum1/1 -> ubalance/1
  Gain/1 -> Sum1/1
  Gain1/1 -> Sum1/2

== system nms_sim_2D_cost/CPG-reflex-synergy controller/Central Pattern Generator ==
  phi out : Inport
  phi right : Inport  Port=2
  Left Central Pattern Generator : Subsystem
  Right Central Pattern Generator : Subsystem
  Outport : Outport
  Outport1 : Outport  Port=2
  wires:
  Right Central Pattern Generator/1(Outport) -> Outport1/1
  Left Central Pattern Generator/1(Outport) -> Outport/1
  phi out/1 -> Left Central Pattern Generator/1(Inport)
  phi right/1 -> Right Central Pattern Generator/1(Inport)

== system nms_sim_2D_cost/CPG-reflex-synergy controller/MN ==
  in : Inport
  Constant : Constant  Value=tau_act_diRusso
  Divide : Product  Inputs=*/
  Integrator : Integrator  InitialCondition=init_exc
  Sum : Sum  Inputs=+-|
  out : Outport  VectorParamsAs1DForOutWhenUnconnected=off
  wires:
  Constant/1 -> Divide/2
  in/1 -> Sum/1
  Integrator/1 -> out/1, Sum/2  "A"
  Divide/1 -> Integrator/1  "dA"
  Sum/1 -> Divide/1

== system nms_sim_2D_cost/CPG-reflex-synergy controller/MN1 ==
  in : Inport
  Constant : Constant  Value=tau_act_diRusso
  Divide : Product  Inputs=*/
  Integrator : Integrator  InitialCondition=init_exc
  Sum : Sum  Inputs=+-|
  out : Outport  VectorParamsAs1DForOutWhenUnconnected=off
  wires:
  Sum/1 -> Divide/1
  Divide/1 -> Integrator/1  "dA"
  Integrator/1 -> Sum/2, out/1  "A"
  in/1 -> Sum/1
  Constant/1 -> Divide/2

== system nms_sim_2D_cost/CPG-reflex-synergy controller/MN10 ==
  in : Inport
  Constant : Constant  Value=tau_act_diRusso
  Divide : Product  Inputs=*/
  Integrator : Integrator  InitialCondition=init_exc
  Sum : Sum  Inputs=+-|
  out : Outport  VectorParamsAs1DForOutWhenUnconnected=off
  wires:
  Constant/1 -> Divide/2
  in/1 -> Sum/1
  Integrator/1 -> out/1, Sum/2  "A"
  Divide/1 -> Integrator/1  "dA"
  Sum/1 -> Divide/1

== system nms_sim_2D_cost/CPG-reflex-synergy controller/MN11 ==
  in : Inport
  Constant : Constant  Value=tau_act_diRusso
  Divide : Product  Inputs=*/
  Integrator : Integrator  InitialCondition=init_exc
  Sum : Sum  Inputs=+-|
  out : Outport  VectorParamsAs1DForOutWhenUnconnected=off
  wires:
  Constant/1 -> Divide/2
  in/1 -> Sum/1
  Integrator/1 -> out/1, Sum/2  "A"
  Divide/1 -> Integrator/1  "dA"
  Sum/1 -> Divide/1

== system nms_sim_2D_cost/CPG-reflex-synergy controller/MN12 ==
  in : Inport
  Constant : Constant  Value=tau_act_diRusso
  Divide : Product  Inputs=*/
  Integrator : Integrator  InitialCondition=init_exc
  Sum : Sum  Inputs=+-|
  out : Outport  VectorParamsAs1DForOutWhenUnconnected=off
  wires:
  Sum/1 -> Divide/1
  Divide/1 -> Integrator/1  "dA"
  Integrator/1 -> Sum/2, out/1  "A"
  in/1 -> Sum/1
  Constant/1 -> Divide/2

== system nms_sim_2D_cost/CPG-reflex-synergy controller/MN13 ==
  in : Inport
  Constant : Constant  Value=tau_act_diRusso
  Divide : Product  Inputs=*/
  Integrator : Integrator  InitialCondition=init_exc
  Sum : Sum  Inputs=+-|
  out : Outport  VectorParamsAs1DForOutWhenUnconnected=off
  wires:
  Constant/1 -> Divide/2
  in/1 -> Sum/1
  Integrator/1 -> out/1, Sum/2  "A"
  Divide/1 -> Integrator/1  "dA"
  Sum/1 -> Divide/1

== system nms_sim_2D_cost/CPG-reflex-synergy controller/MN14 ==
  in : Inport
  Constant : Constant  Value=tau_act_diRusso
  Divide : Product  Inputs=*/
  Integrator : Integrator  InitialCondition=init_exc
  Sum : Sum  Inputs=+-|
  out : Outport  VectorParamsAs1DForOutWhenUnconnected=off
  wires:
  Sum/1 -> Divide/1
  Divide/1 -> Integrator/1  "dA"
  Integrator/1 -> Sum/2, out/1  "A"
  in/1 -> Sum/1
  Constant/1 -> Divide/2

== system nms_sim_2D_cost/CPG-reflex-synergy controller/MN15 ==
  in : Inport
  Constant : Constant  Value=tau_act_diRusso
  Divide : Product  Inputs=*/
  Integrator : Integrator  InitialCondition=init_exc
  Sum : Sum  Inputs=+-|
  out : Outport  VectorParamsAs1DForOutWhenUnconnected=off
  wires:
  Sum/1 -> Divide/1
  Divide/1 -> Integrator/1  "dA"
  Integrator/1 -> Sum/2, out/1  "A"
  in/1 -> Sum/1
  Constant/1 -> Divide/2

== system nms_sim_2D_cost/CPG-reflex-synergy controller/MN16 ==
  in : Inport
  Constant : Constant  Value=tau_act_diRusso
  Divide : Product  Inputs=*/
  Integrator : Integrator  InitialCondition=init_exc
  Sum : Sum  Inputs=+-|
  out : Outport  VectorParamsAs1DForOutWhenUnconnected=off
  wires:
  Constant/1 -> Divide/2
  in/1 -> Sum/1
  Integrator/1 -> out/1, Sum/2  "A"
  Divide/1 -> Integrator/1  "dA"
  Sum/1 -> Divide/1

== system nms_sim_2D_cost/CPG-reflex-synergy controller/MN17 ==
  in : Inport
  Constant : Constant  Value=tau_act_diRusso
  Divide : Product  Inputs=*/
  Integrator : Integrator  InitialCondition=init_exc
  Sum : Sum  Inputs=+-|
  out : Outport  VectorParamsAs1DForOutWhenUnconnected=off
  wires:
  Sum/1 -> Divide/1
  Divide/1 -> Integrator/1  "dA"
  Integrator/1 -> Sum/2, out/1  "A"
  in/1 -> Sum/1
  Constant/1 -> Divide/2

== system nms_sim_2D_cost/CPG-reflex-synergy controller/MN2 ==
  in : Inport
  Constant : Constant  Value=tau_act_diRusso
  Divide : Product  Inputs=*/
  Integrator : Integrator  InitialCondition=init_exc
  Sum : Sum  Inputs=+-|
  out : Outport  VectorParamsAs1DForOutWhenUnconnected=off
  wires:
  Sum/1 -> Divide/1
  Divide/1 -> Integrator/1  "dA"
  Integrator/1 -> Sum/2, out/1  "A"
  in/1 -> Sum/1
  Constant/1 -> Divide/2

== system nms_sim_2D_cost/CPG-reflex-synergy controller/MN3 ==
  in : Inport
  Constant : Constant  Value=tau_act_diRusso
  Divide : Product  Inputs=*/
  Integrator : Integrator  InitialCondition=init_exc
  Sum : Sum  Inputs=+-|
  out : Outport  VectorParamsAs1DForOutWhenUnconnected=off
  wires:
  Constant/1 -> Divide/2
  in/1 -> Sum/1
  Integrator/1 -> out/1, Sum/2  "A"
  Divide/1 -> Integrator/1  "dA"
  Sum/1 -> Divide/1

== system nms_sim_2D_cost/CPG-reflex-synergy controller/MN4 ==
  in : Inport
  Constant : Constant  Value=tau_act_diRusso
  Divide : Product  Inputs=*/
  Integrator : Integrator  InitialCondition=init_exc
  Sum : Sum  Inputs=+-|
  out : Outport  VectorParamsAs1DForOutWhenUnconnected=off
  wires:
  Sum/1 -> Divide/1
  Divide/1 -> Integrator/1  "dA"
  Integrator/1 -> Sum/2, out/1  "A"
  in/1 -> Sum/1
  Constant/1 -> Divide/2

== system nms_sim_2D_cost/CPG-reflex-synergy controller/MN5 ==
  in : Inport
  Constant : Constant  Value=tau_act_diRusso
  Divide : Product  Inputs=*/
  Integrator : Integrator  InitialCondition=init_exc
  Sum : Sum  Inputs=+-|
  out : Outport  VectorParamsAs1DForOutWhenUnconnected=off
  wires:
  Constant/1 -> Divide/2
  in/1 -> Sum/1
  Integrator/1 -> out/1, Sum/2  "A"
  Divide/1 -> Integrator/1  "dA"
  Sum/1 -> Divide/1

== system nms_sim_2D_cost/CPG-reflex-synergy controller/MN6 ==
  in : Inport
  Constant : Constant  Value=tau_act_diRusso
  Divide : Product  Inputs=*/
  Integrator : Integrator  InitialCondition=init_exc
  Sum : Sum  Inputs=+-|
  out : Outport  VectorParamsAs1DForOutWhenUnconnected=off
  wires:
  Constant/1 -> Divide/2
  in/1 -> Sum/1
  Integrator/1 -> out/1, Sum/2  "A"
  Divide/1 -> Integrator/1  "dA"
  Sum/1 -> Divide/1

== system nms_sim_2D_cost/CPG-reflex-synergy controller/MN7 ==
  in : Inport
  Constant : Constant  Value=tau_act_diRusso
  Divide : Product  Inputs=*/
  Integrator : Integrator  InitialCondition=init_exc
  Sum : Sum  Inputs=+-|
  out : Outport  VectorParamsAs1DForOutWhenUnconnected=off
  wires:
  Sum/1 -> Divide/1
  Divide/1 -> Integrator/1  "dA"
  Integrator/1 -> Sum/2, out/1  "A"
  in/1 -> Sum/1
  Constant/1 -> Divide/2

== system nms_sim_2D_cost/CPG-reflex-synergy controller/MN8 ==
  in : Inport
  Constant : Constant  Value=tau_act_diRusso
  Divide : Product  Inputs=*/
  Integrator : Integrator  InitialCondition=init_exc
  Sum : Sum  Inputs=+-|
  out : Outport  VectorParamsAs1DForOutWhenUnconnected=off
  wires:
  Constant/1 -> Divide/2
  in/1 -> Sum/1
  Integrator/1 -> out/1, Sum/2  "A"
  Divide/1 -> Integrator/1  "dA"
  Sum/1 -> Divide/1

== system nms_sim_2D_cost/CPG-reflex-synergy controller/MN9 ==
  in : Inport
  Constant : Constant  Value=tau_act_diRusso
  Divide : Product  Inputs=*/
  Integrator : Integrator  InitialCondition=init_exc
  Sum : Sum  Inputs=+-|
  out : Outport  VectorParamsAs1DForOutWhenUnconnected=off
  wires:
  Sum/1 -> Divide/1
  Divide/1 -> Integrator/1  "dA"
  Integrator/1 -> Sum/2, out/1  "A"
  in/1 -> Sum/1
  Constant/1 -> Divide/2
